simulink model "vdynblksskidpad"  (R2023a)
settings: Solver=ode23tb  StartTime=0.0  StopTime=35  MaxStep=.02  RelTol=1e-1  AbsTol=5e-3
model workspace (MAT data in the model file):
  Eng : object (value not decoded)
  SteerLim = 60
  TrackPoints = [-15 -12 -9 -6 -3 5.58745102111e-16 2.81978007367 5.36354042717 7.38228007367 8.67839071119 9.125 8.67839071119 ... (270 elements, 90x3)]
  Trans : object (value not decoded)
  Ts = 0.02
  VEH : object (value not decoded)
symbols that are objects in the model workspace (value not decoded): Eng, Trans, VEH
undefined symbols (not defined in the file or in its folder): BdyFrm, InertFrm
libraries: autolibsharedcoupling x11, simulink x8, autolibshareddiff x5, sim3dlib x4, autolibutils x3, vehdynlibtirecommon x3, sharedtransform x3, vehdynlibdriver x2, sim3dautolib x2, vehdynlibviscommon x2, visionanalysis x1, vehdynlibtire x1
(part 3 of 3)

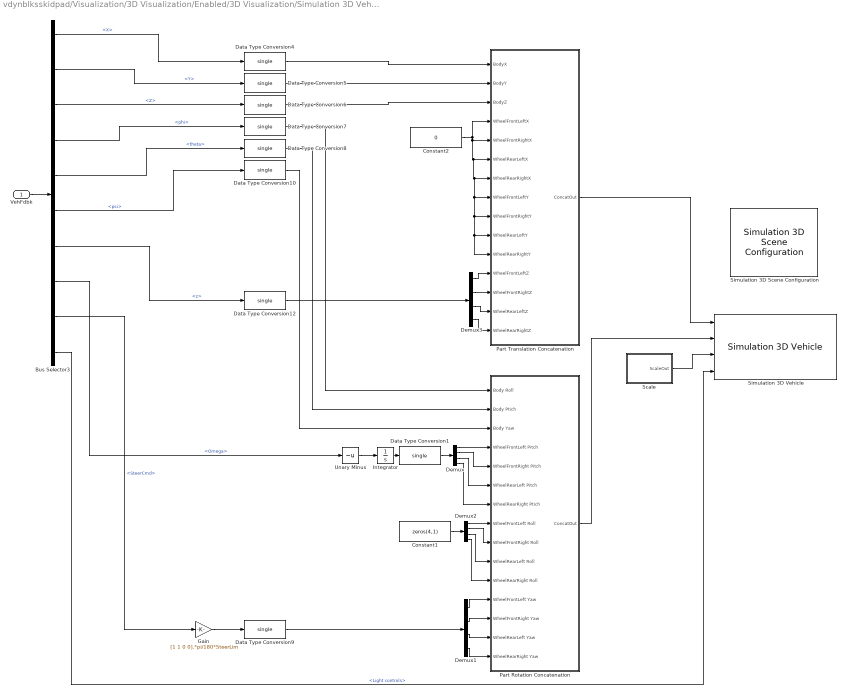
== system vdynblksskidpad/Visualization/3D Visualization/Enabled/3D Visualization/Simulation 3D Vehicle ==
  VehFdbk : Inport
  Bus Selector3 : BusSelector  OutputSignals=VehFdbk.InertFrm.Cg.Disp.X,VehFdbk.InertFrm.Cg.Disp.Y,VehFdbk.InertFrm.Cg.Disp.Z,VehFdbk.InertFrm.Cg.Ang.phi,VehFdbk.InertFrm.Cg.Ang.theta,VehFdbk.InertFrm.Cg.Ang.psi,VehFdbk.Wheels.z,VehFdbk.Wheels.Omega,Driver.SteerCmd,Driver.Light controls
  Constant1 : Constant  Value=zeros(4,1)  OutDataTypeStr=single
  Constant2 : Constant  Value=0  OutDataTypeStr=single
  Data Type Conversion{1,4..10,12} (9 alike) : DataTypeConversion  OutDataTypeStr=single  SaturateOnIntegerOverflow=off  RndMeth=Floor
  Demux{,1..3} (4 alike) : Demux
  Gain : Gain  Gain=[1 1 0 0].*pi/180*SteerLim
  Integrator : Integrator  WrapState=on  WrappedStateUpperValue=2*pi  WrappedStateLowerValue=0  ZeroCross=off
  Part Rotation Concatenation : Subsystem
  Part Translation Concatenation : Subsystem
  Scale : Subsystem
  Simulation 3D Scene Configuration : sim3dlib/Simulation 3D Scene Configuration  Priority=0  ProjectFormat=Default Scenes  SceneDesc=Open surface  ProjectName=C:\Program Files\MATLAB\R2023b\toolbox\shared\sim3d_projects\automotive_project_windows\UE\WindowsNoEditor\VehicleSimulation.exe  ScenePath=/Game/Maps/BlackLake  EnableOpenDRIVE=off  vehTagList={'Scene Origin';'Sim3dActor1';'SimulinkVehicle3'}  vehTag=SimulinkVehicle3  FreeCameraInitialTranslation=[0, 0, 0]  FreeCameraDefaultInitialTranslation=[-6, 0, 2]  FreeCameraInitialRotation=[0, 0, 0]  FreeCameraDefaultInitialRotation=[0, -15, 0]  OpVisEn=off  Ts=Ts  EnableWindow=on  EnableRemoteAccess=off  EnableWeather=off  SunAltitude=40.0  SunAzimuth=90  clouds=10  wind=1  fog=0  rain=0  EnableGeospatial=off  OriginHeight=200  OriginLatitude=40.744652  OriginLongitude=-73.988864  MapStyle=Aerial  AdditionalAssetIDs=[]  UseAdvancedSunSky=off  SolarTime=11  TimeZone=-5  Day=21  Month=9  Year=2022  UseDaylightSavingTime=on  DSTStartDay=10  DSTStartMonth=3  DSTEndDay=3  DSTEndMonth=11  DSTSwitchHour=2  sensorTag=MainCamera3  sensorId=3  sensorName=MainCamera3  mountLoc=Origin  offsetFlag=off  tmountOffset=[0, 0, 0]  rmountOffset=[0, 0, 0]  HorizontalResolution=1280  VerticalResolution=720  HorizontalFOV=60  mountPoint=[0 0 0]  mountOrientation=[0 0 0]  aMode=2  ID=3  GeoTrigger=Inactive
      settings: LibrarySourceBlock=vdynlib/Vehicle Scenarios/Sim3D/Sim3D Core/Simulation 3D Scene Configuration
  Simulation 3D Vehicle : sim3dautolib/Simulation 3D Vehicle  Priority=-1  PassVehMesh=Formula student vehicle  MeshPath=/MathWorksSimulation/Vehicles/Muscle/Meshes/SK_MuscleCar.SK_MuscleCar  VehColor=Red  ActorName=SimulinkVehicle3  VehLightsControl=on  HeadlightColor=[ 1, 1, 1 ]  HighBeamIntensity=100000  LowBeamIntensity=60000  HighBeamConeAngle=1.22  LowBeamConeAngle=1.22  LeftHeadlightOrientation=[ 0, 0 ]  RightHeadlightOrientation=[ 0, 0 ]  BrakelightIntensity=500  ReverselightIntensity=500  SignallightIntensity=500  SignallightPeriod=1  SignalPulseWidth=50  Translation=[ VEH.InitialLongPosition, VEH.InitialLatPosition, VEH.InitialVertPosition *0; zeros(4,3)]  Rotation=[VEH.InitialRollAngle VEH.InitialPitchAngle VEH.InitialYawAngle; zeros( 4, 3 )]  Scale=ones( 5, 3 )  SampleTime=Ts  ActorType=SimulinkVehicle  ID=3  aMode=2  ActorTag=SimulinkVehicle3
      settings: LibrarySourceBlock=vdynlib/Vehicle Scenarios/Sim3D/Sim3D Vehicle/Components/Simulation 3D Vehicle
  Unary Minus : UnaryMinus
  wires:
  Bus Selector3/6 -> Data Type Conversion10/1  "<psi>"
  Bus Selector3/10 -> Simulation 3D Vehicle/4  "<Light controls>"
  Bus Selector3/2 -> Data Type Conversion5/1  "<Y>"
  VehFdbk/1 -> Bus Selector3/1
  Bus Selector3/1 -> Data Type Conversion4/1  "<X>"
  Data Type Conversion10/1 -> Part Rotation Concatenation/3(Body Yaw)
  Data Type Conversion5/1 -> Part Translation Concatenation/2(BodyY)
  Constant2/1 -> Part Translation Concatenation/5(WheelFrontRightX), Part Translation Concatenation/6(WheelRearLeftX), Part Translation Concatenation/7(WheelRearRightX), Part Translation Concatenation/8(WheelFrontLeftY), Part Translation Concatenation/9(WheelFrontRightY), Part Translation Concatenation/10(WheelRearLeftY), Part Translation Concatenation/11(WheelRearRightY), Part Translation Concatenation/4(WheelFrontLeftX)
  Data Type Conversion8/1 -> Part Rotation Concatenation/2(Body Ptich)
  Demux2/2 -> Part Rotation Concatenation/9(WheelFrontRight Roll)
  Demux1/3 -> Part Rotation Concatenation/14(WheelRearLeft Yaw)
  Demux/3 -> Part Rotation Concatenation/6(WheelRearLeft Pitch)
  Data Type Conversion9/1 -> Demux1/1
  Demux1/2 -> Part Rotation Concatenation/13(WheelFrontRight Yaw)
  Demux/2 -> Part Rotation Concatenation/5(WheelFrontRight Pitch)
  Demux2/3 -> Part Rotation Concatenation/10(WheelRearLeft Roll)
  Bus Selector3/5 -> Data Type Conversion8/1  "<theta>"
  Data Type Conversion7/1 -> Part Rotation Concatenation/1(Body Roll)
  Demux3/2 -> Part Translation Concatenation/13(WheelFrontRightZ)
  Data Type Conversion4/1 -> Part Translation Concatenation/1(BodyX)
  Integrator/1 -> Data Type Conversion1/1
  Demux2/1 -> Part Rotation Concatenation/8(WheelFrontLeft Roll)
  Demux1/4 -> Part Rotation Concatenation/15(WheelRearRight Yaw)
  Demux3/4 -> Part Translation Concatenation/15(WheelRearRightZ)
  Bus Selector3/4 -> Data Type Conversion7/1  "<phi>"
  Bus Selector3/7 -> Data Type Conversion12/1  "<z>"
  Bus Selector3/8 -> Unary Minus/1  "<Omega>"
  Data Type Conversion1/1 -> Demux/1
  Constant1/1 -> Demux2/1
  Demux3/3 -> Part Translation Concatenation/14(WheelRearLeftZ)
  Part Rotation Concatenation/1(ConcatOut) -> Simulation 3D Vehicle/2
  Demux3/1 -> Part Translation Concatenation/12(WheelFrontLeftZ)
  Part Translation Concatenation/1(ConcatOut) -> Simulation 3D Vehicle/1
  Demux/1 -> Part Rotation Concatenation/4(WheelFrontLeft Pitch)
  Demux1/1 -> Part Rotation Concatenation/12(WheelFrontLeft Yaw)
  Data Type Conversion6/1 -> Part Translation Concatenation/3(BodyZ)
  Unary Minus/1 -> Integrator/1
  Demux/4 -> Part Rotation Concatenation/7(WheelRearRight Ptich)
  Demux2/4 -> Part Rotation Concatenation/11(WheelRearRight Roll)
  Data Type Conversion12/1 -> Demux3/1
  Scale/1(ScaleOut) -> Simulation 3D Vehicle/3
  Bus Selector3/3 -> Data Type Conversion6/1  "<Z>"
  Bus Selector3/9 -> Gain/1  "<SteerCmd>"
  Gain/1 -> Data Type Conversion9/1

== system vdynblksskidpad/Visualization/3D Visualization/Enabled/Cones/Disabled ==

== system vdynblksskidpad/Visualization/3D Visualization/Enabled/Cones/Enabled ==
  Simulation 3D Actor : sim3dlib/Simulation 3D Actor  ActorName=Sim3dActor1  ParentName=Scene Origin  Operation=Create at setup  InitScriptText=|  SampleTime=Ts  Translation=single([0 0 0])  Rotation=single([0 0 0])  Scale=single([1 1 1])  aMode=5  ActorTag=Sim3dActor1  ActorType=Sim3dActor  ID=1
      | entryWidth =3.453;
      | conesZ0 = 0;
      | entryConesLoc = [entryWidth/2 -12;...
      |                  -entryWidth/2 -12;...
      |                  -entryWidth/2 -10;...
      |                  entryWidth/2 -10];
      | entryConesLoc= fliplr(entryConesLoc); % account for game engine coords
      | rightInnerRingLoc = [entryWidth/2 0;...%1
      |                   4.58/2 -2.834;...%2
      |                   7.787/2 -5.231;...%3
      |                   12.588/2 -6.835;...%4
      |                   18.25/2 -7.398;...%5
      |                   23.912/2 -6.835;...%6
      |                   28.713/2 -5.231;...%7
      |                   31.92/2 -2.834;...%8
      |                   33.047/2 0;...%9
      |                   31.92/2 2.834;...%10
      |                   28.713/2 5.231;...%11
      |                   23.912/2 6.835;...%12
      |                   18.25/2 7.398;...%13
      |                   12.588/2 6.835;...%14
      |                   7.787/2 5.231;...%15
      |                   4.58/2 2.834;...%16    
      |                   ];
      | rightInnerRingLoc = fliplr(rightInnerRingLoc);
      | leftInnerRingLoc = rightInnerRingLoc.*[1 -1];
      | rightOutterRingLoc = [entryWidth/2 7.939;...% right side entry to exit zone
      |                       9.945/2 10.026;...
      |                       18.25/2 10.852;...
      |                       26.555/2 10.026;...
      |                       33.596/2 7.673;...
      |                       38.301/2 4.153;...
      |                       39.953/2 0;...
      |                       38.301/2 -4.153;...
      |                       33.596/2 -7.673;...
      |                       26.555/2 -10.026;...
      |                       18.25/2 -10.852;...
      |                       9.945/2 -10.026;...                      
      |                       entryWidth/2 -7.939;...% right side after entry zone                      
      |                       ];
      | rightOutterRingLoc = fliplr(rightOutterRingLoc);
      | leftOutterRingLoc = rightOutterRingLoc.*[1 -1];
      | 
      | exitConesLoc = [entryWidth/2 16;...
      |                  -entryWidth/2 16;...
      |                  entryWidth/2-1 16;...
      |                  -entryWidth/2+1 16;...
      |                  -entryWidth/2 14;...
      |                  entryWidth/2 14;...
      |                  -entryWidth/2 12;...
      |                  entryWidth/2 12;...
      |                  -entryWidth/2 10;...
      |                  entryWidth/2 10];
      | exitConesLoc= fliplr(exitConesLoc); % account for game engine coords
      | 
      | timeConesLoc = fliplr([entryWidth/2 .5;...
      |                  -entryWidth/2 .5;...
      |                  entryWidth/2 -.5;...
      |                  -entryWidth/2 -.5]);
      | 
      | blueCones = [rightOutterRingLoc; leftInnerRingLoc];
      | yellowCones = [rightInnerRingLoc; leftOutterRingLoc];
      | smallOrangeCones = [entryConesLoc; exitConesLoc];
      | largeOrangeCones = timeConesLoc;
      | 
      | skidSurface = sim3d.Actor('ActorName','BaseSurface');
      | skidSurface.createShape('box',[45,45,+0.03]);
      | skidSurface.Color = [68 68 71]./100;
      | skidSurface.Translation = [0 0 0]; 
      | skidSurface.Texture = fullfile(pwd,"vdynskidpad.png"); 
      | skidSurface.TextureTransform.Scale = [1 1];
      | skidSurface.TextureTransform.Angle = 0;
      | skidSurface.Shininess = 0;
      | skidSurface.Transparency = 0;
      | skidSurface.TextureMapping.Blend = 1;
      | skidSurface.TextureMapping.Roughness = .8;
      | World.add(skidSurface,Actor);
      | 
      | nCones = length(largeOrangeCones);
      | for coneNum = 1:nCones    
      |     coneName = "LCone_" + num2str(coneNum);
      |     conLoc = [largeOrangeCones(coneNum,:) conesZ0];
      |     cone = sim3d.Actor('ActorName',coneName,'Mesh','/Game/Environment/Industrial/Props/Cone/Mesh/SM_Cone.SM_Cone',...
      |         'Mobility', sim3d.utils.MobilityTypes.Movable,...
      |         'SimulatePhysics', true,...
      |         'Translation',conLoc,...
      |         'EnableGravity', true);    
      |     %cone.Shadows = true;
      |     World.add(cone,Actor);
      | end
      | 
      | smallCones = [blueCones; yellowCones; smallOrangeCones]; 
      | for coneNum = 1:length(smallCones)    
      |     coneName = "sCone_" + num2str(coneNum);
      |     conLoc = [smallCones(coneNum,:) conesZ0];
      |     cone = sim3d.Actor('ActorName',coneName,'Mesh','/Game/Environment/Industrial/Props/Cone/Mesh/SM_Cone.SM_Cone',...
      |         'Mobility', sim3d.utils.MobilityTypes.Movable,...
      |         'SimulatePhysics', true,...
      |         'Translation',conLoc,...
      |         'EnableGravity', true,...
      |         'Scale',ones(1,3).*325/500);    
      |     cone.Color= [102 140 204]./255;
      |     World.add(cone,Actor);
      | end
      settings: LibrarySourceBlock=sl3dlib/Simulation 3D/Simulation 3D Actor
  Terminator : Terminator
  wires:
  Simulation 3D Actor/1 -> Terminator/1

== system vdynblksskidpad/Formula Student Vehicle/Simulink Physics - 7DOF/Powertrain & Driveline/Brakes and Wheels/Tire2Veh/Wheel Angles ==
  Front : Inport
  Camber : Inport  Port=2
  Constant : Constant  Value=zeros(4,1)
  Reshape : Reshape  OutputDimensionality=Row vector (2-D)
  Reshape1 : Reshape  OutputDimensionality=Row vector (2-D)
  Reshape2 : Reshape  OutputDimensionality=Row vector (2-D)
  Vector Concatenate3 : Concatenate  NumInputs=3  Mode=Multidimensional array
  Vehicle : Outport  VectorParamsAs1DForOutWhenUnconnected=off
  wires:
  Reshape/1 -> Vector Concatenate3/3
  Reshape2/1 -> Vector Concatenate3/2
  Vector Concatenate3/1 -> Vehicle/1
  Reshape1/1 -> Vector Concatenate3/1
  Front/1 -> Reshape/1
  Camber/1 -> Reshape1/1
  Constant/1 -> Reshape2/1

== system vdynblksskidpad/Formula Student Vehicle/Simulink Physics - 7DOF/Powertrain & Driveline/Brakes and Wheels/Tire2Veh/Wheel to Body Transform ==
  Forces : Inport  PortDimensions=[3,1]  Partition=on  PartitionDimension=2  PartitionWidth=1  PartitionOffset=0
  WheelAngles : Inport  Port=2  Partition=on  PartitionDimension=2  PartitionWidth=1  PartitionOffset=0
  Constant : Constant  Value=[pi;0;0]
  Demux1 : Demux  Outputs=3
  Divide1 : Product  Inputs=***  Multiplication=Matrix(*)
  For Each : ForEach  DisableCoverage=on
  Rotation Angles to Direction Cosine Matrix : sharedtransform/Rotation Angles to Direction Cosine Matrix  rotationOrder=ZYX  aMode=2
  Rotation Angles to Direction Cosine Matrix1 : sharedtransform/Rotation Angles to Direction Cosine Matrix  rotationOrder=ZYX  aMode=2
  Selector : Selector  InputPortWidth=3  IndexOptions=Index vector (dialog)  Indices=[3 2 1]  OutputSizes=1
  Selector1 : Selector  InputPortWidth=3  IndexOptions=Index vector (dialog)  Indices=[3 2 1]  OutputSizes=1
  Transpose : Math  Operator=transpose
  Fx : Outport  ConcatenationDimension=1  VectorParamsAs1DForOutWhenUnconnected=off
  Fy : Outport  Port=2  ConcatenationDimension=1  VectorParamsAs1DForOutWhenUnconnected=off
  Fz : Outport  Port=3  ConcatenationDimension=1  VectorParamsAs1DForOutWhenUnconnected=off
  wires:
  Demux1/1 -> Fx/1
  Demux1/2 -> Fy/1
  Demux1/3 -> Fz/1
  Rotation Angles to Direction Cosine Matrix/1 -> Transpose/1
  Forces/1 -> Divide1/3
  WheelAngles/1 -> Selector/1
  Selector/1 -> Rotation Angles to Direction Cosine Matrix/1
  Rotation Angles to Direction Cosine Matrix1/1 -> Divide1/2
  Divide1/1 -> Demux1/1
  Selector1/1 -> Rotation Angles to Direction Cosine Matrix1/1
  Constant/1 -> Selector1/1
  Transpose/1 -> Divide1/1

== system vdynblksskidpad/Formula Student Vehicle/Simulink Physics - 7DOF/Powertrain & Driveline/Brakes and Wheels/Veh2Tire/Wheel to Body Transform ==
  VelVeh : Inport  Partition=on  PartitionDimension=2  PartitionWidth=1  PartitionOffset=0
  WhlAng : Inport  Port=2  Partition=on  PartitionDimension=2  PartitionWidth=1  PartitionOffset=0
  Demux1 : Demux  Outputs=3
  Divide1 : Product  Inputs=**  Multiplication=Matrix(*)
  For Each : ForEach  DisableCoverage=on
  Rotation Angles to Direction Cosine Matrix : sharedtransform/Rotation Angles to Direction Cosine Matrix  rotationOrder=ZYX  aMode=2
  Selector : Selector  InputPortWidth=3  IndexOptions=Index vector (dialog)  Indices=[3 2 1]  OutputSizes=1
  xdotWheel : Outport  ConcatenationDimension=1  VectorParamsAs1DForOutWhenUnconnected=off
  ydotWheel : Outport  Port=2  ConcatenationDimension=1  VectorParamsAs1DForOutWhenUnconnected=off
  zdotWheel : Outport  Port=3  ConcatenationDimension=1  VectorParamsAs1DForOutWhenUnconnected=off
  wires:
  Divide1/1 -> Demux1/1
  Demux1/1 -> xdotWheel/1
  Demux1/2 -> ydotWheel/1
  Demux1/3 -> zdotWheel/1
  Rotation Angles to Direction Cosine Matrix/1 -> Divide1/1
  VelVeh/1 -> Divide1/2
  WhlAng/1 -> Selector/1
  Selector/1 -> Rotation Angles to Direction Cosine Matrix/1

== system vdynblksskidpad/Formula Student Vehicle/Simulink Physics - 7DOF/Powertrain & Driveline/Powertrain/Transmission/Ideal ==
  GearCmd : Inport
  EngTrq : Inport  Port=2
  PropShftSpd : Inport  Port=3
  Ideal Fixed Gear Transmission : autolibsharedtransfixedgear/Ideal Fixed Gear Transmission  VariantControl=0  TransEffModelPopup=Gear only  gearInterp=Linear point-slope  G=Trans.GearNums  Trq_bpts=[25, 50, 75, 100, 150, 200, 250]  omega_bpts=[52.4 78.5 105 131 157 183 209 262 314 419 524]  Temp_bpts=[313 358]  N=Trans.GearRatios  Jout=Trans.Inertias  bout=Trans.DampingCoeffs  eta=Trans.Efficiencies  eta_tbl=reshape([0.53 0.71 0.77 0.79 0.82 0.82 0.82 0.5 0.7 0.77 0.79 0.82 0.82 0.82 0.54 0.72 0.78 0.81 0.83 0.82 0.82 0.56 0.73 0.79 0.81 0.84 0.82 0.82 0.58 0.74 0.79 0.82 0.84 0.82 0.82 0.57 0.74 0.79 0.82 0.84 0.82 0.82 0.58 0.74 0.79 0.82 0.84 0.82 0.82 0.58 0.74 0.79 0.82 0.84 0.82 0.82 0.57 0.74 0.8 0.82 0.85 0.82 0.82 0.55 0.73 0.78 0.81 0.84 0.82 0.82 0.51 0.71 0.77 0.81 0.84 0.82 0.82 0.53 0.71 0.77 0.79 0.82 0.82 0.82 0.5 0.7 0.77 0.79 0.82 0.82 0.82 0.54 0.72 0.78 0.81 0.83 0.82 0.82 0.56 0.73 0.79 0.81 0.84 0.82 0.82 0.58 0.74 0.79 0.82 0.84 0.82 0.82 0.57 0.74 0.79 0.82 0.84 0.82 0.82 0.58 0.74 0.79 0.82 0.84 0.82 0.82 0.58 0.74 0.79 0.82 0.84 0.82 0.82 0.57 0.74 0.8 0.82 0.85 0.82 0.82 0.55 0.73 0.78 0.81 0.84 0.82 0.82 0.51 0.71 0.77 0.81 0.84 0.82 0.82 0.53 0.71 0.77 0.79 0.82 0.82 0.82 0.5 0.7 0.77 0.79 0.82 0.82 0.82 0.54 0.72 0.78 0.81 0.83 0.82 0.82 0.56 0.73 0.79 0.81 0.84 0.82 0.82 0.58 0.74 0.79 0.82 0.84 0.82 0.82 0.57 0.74 0.79 0.82 0.84 0.82 0.82 0.58 0.74 0.79 0.82 0.84 0.82 0.82 0.58 0.74 0.79 0.82 0.84 0.82 0.82 0.57 0.74 0.8 0.82 0.85 0.82 0.82 0.55 0.73 0.78 0.81 0.84 0.82 0.82 0.51 0.71 0.77 0.81 0.84 0.82 0.82 0.7 0.79 0.82 0.83 0.84 0.84 0.84 0.63 0.76 0.8 0.82 0.83 0.84 0.84 0.58 0.74 0.79 0.81 0.83 0.84 0.84 0.58 0.74 0.79 0.81 0.83 0.84 0.84 0.58 0.74 0.79 0.81 0.84 0.84 0.84 0.57 0.73 0.78 0.81 0.84 0.85 0.84 0.57 0.73 0.79 0.81 0.84 0.85 0.84 0.56 0.73 0.78 0.81 0.83 0.85 0.84 0.55 0.73 0.78 0.81 0.84 0.85 0.84 0.52 0.71 0.77 0.8 0.83 0.85 0.84 0.48 0.69 0.76 0.79 0.83 0.84 0.84 0.64 0.76 0.8 0.81 0.83 0.84 0.84 0.56 0.73 0.78 0.8 0.83 0.84 0.84 0.54 0.71 0.77 0.8 0.82 0.84 0.84 0.53 0.71 0.77 0.8 0.83 0.84 0.84 0.51 0.71 0.77 0.8 0.83 0.84 0.85 0.52 0.7 0.77 0.8 0.83 0.84 0.85 0.51 0.71 0.76 0.79 0.83 0.84 0.85 0.5 0.69 0.76 0.79 0.82 0.84 0.85 0.45 0.68 0.75 0.78 0.82 0.84 0.85 0.43 0.67 0.74 0.78 0.81 0.83 0.84 0.38 0.63 0.71 0.75 0.8 0.82 0.83 0.65 0.79 0.84 0.85 0.88 0.89 0.89 0.56 0.75 0.81 0.83 0.86 0.88 0.89 0.52 0.72 0.79 0.83 0.86 0.88 0.88 0.51 0.72 0.79 0.83 0.86 0.88 0.89 0.49 0.71 0.78 0.82 0.86 0.88 0.89 0.47 0.7 0.78 0.82 0.86 0.87 0.88 0.45 0.69 0.77 0.81 0.85 0.87 0.88 0.4 0.67 0.75 0.8 0.84 0.86 0.88 0.3 0.64 0.73 0.78 0.83 0.86 0.87 0.17 0.55 0.67 0.73 0.8 0.83 0.85 0.089 0.45 0.61 0.69 0.77 0.81 0.83 0.61 0.75 0.82 0.84 0.87 0.87 0.88 0.54 0.73 0.8 0.82 0.86 0.87 0.88 0.51 0.71 0.79 0.82 0.86 0.87 0.88 0.52 0.72 0.79 0.82 0.86 0.87 0.89 0.52 0.72 0.8 0.83 0.86 0.88 0.89 0.53 0.72 0.79 0.82 0.86 0.87 0.89 0.5 0.7 0.78 0.82 0.86 0.88 0.88 0.46 0.69 0.77 0.81 0.85 0.87 0.88 0.4 0.67 0.75 0.8 0.83 0.86 0.88 0.33 0.64 0.73 0.78 0.83 0.85 0.87 0.33 0.64 0.73 0.78 0.83 0.85 0.87 0.78 0.85 0.87 0.88 0.89 0.89 0.89 0.73 0.83 0.86 0.88 0.89 0.89 0.89 0.72 0.83 0.86 0.88 0.89 0.89 0.89 0.72 0.83 0.87 0.89 0.9 0.89 0.89 0.72 0.83 0.87 0.88 0.9 0.89 0.89 0.71 0.83 0.87 0.88 0.9 0.89 0.89 0.71 0.83 0.86 0.88 0.9 0.89 0.89 0.7 0.82 0.86 0.88 0.9 0.89 0.89 0.69 0.82 0.86 0.88 0.9 0.89 0.89 0.67 0.81 0.86 0.88 0.9 0.89 0.89 0.63 0.79 0.85 0.87 0.89 0.89 0.89 0.78 0.85 0.87 0.88 0.89 0.89 0.89 0.73 0.83 0.86 0.88 0.89 0.89 0.89 0.72 0.83 0.86 0.88 0.89 0.89 0.89 0.72 0.83 0.87 0.89 0.9 0.89 0.89 0.72 0.83 0.87 0.88 0.9 0.89 0.89 0.71 0.83 0.87 0.88 0.9 0.89 0.89 0.71 0.83 0.86 0.88 0.9 0.89 0.89 0.7 0.82 0.86 0.88 0.9 0.89 0.89 0.69 0.82 0.86 0.88 0.9 0.89 0.89 0.67 0.81 0.86 0.88 0.9 0.89 0.89 0.63 0.79 0.85 0.87 0.89 0.89 0.89 0.78 0.85 0.87 0.88 0.89 0.89 0.89 0.73 0.83 0.86 0.88 0.89 0.89 0.89 0.72 0.83 0.86 0.88 0.89 0.89 0.89 0.72 0.83 0.87 0.89 0.9 0.89 0.89 0.72 0.83 0.87 0.88 0.9 0.89 0.89 0.71 0.83 0.87 0.88 0.9 0.89 0.89 0.71 0.83 0.86 0.88 0.9 0.89 0.89 0.7 0.82 0.86 0.88 0.9 0.89 0.89 0.69 0.82 0.86 0.88 0.9 0.89 0.89 0.67 0.81 0.86 0.88 0.9 0.89 0.89 0.63 0.79 0.85 0.87 0.89 0.89 0.89 0.82 0.87 0.88 0.89 0.89 0.89 0.89 0.81 0.87 0.89 0.89 0.9 0.9 0.89 0.76 0.85 0.87 0.89 0.9 0.89 0.89 0.72 0.83 0.86 0.88 0.89 0.89 0.89 0.72 0.83 0.86 0.88 0.89 0.9 0.89 0.71 0.82 0.86 0.88 0.89 0.9 ...(+1314 chars))  G_o=0  omega_o=0  omegaN_o=0  tau_s=Trans.ShiftTau  maxAbsSpd=5e3  aMode=2
      settings: LibrarySourceBlock=vdynlib/Powertrain/Transmission/Ideal Fixed Gear Transmission
  Prop Shaft : autolibsharedcoupling/Torsional Compliance  port_config=Simulink  extInfo=off  k=5e3  b=10  theta_o=0  domega_o=0  omega_c=100  blkID=0  aMode=2
      settings: LibrarySourceBlock=vdynlib/Powertrain/Drivetrain/Couplings/Torsional Compliance
  Unit Conversion : UnitConversion
  Info : Outport  VectorParamsAs1DForOutWhenUnconnected=off
  EngSpd : Outport  Port=2  VectorParamsAs1DForOutWhenUnconnected=off
  DrvShfTrq : Outport  Port=3  VectorParamsAs1DForOutWhenUnconnected=off
  wires:
  Ideal Fixed Gear Transmission/2 -> Unit Conversion/1
  GearCmd/1 -> Ideal Fixed Gear Transmission/1
  Ideal Fixed Gear Transmission/1 -> Info/1
  PropShftSpd/1 -> Prop Shaft/2
  Ideal Fixed Gear Transmission/3 -> Prop Shaft/1
  Prop Shaft/2 -> DrvShfTrq/1
  Prop Shaft/1 -> Ideal Fixed Gear Transmission/3
  EngTrq/1 -> Ideal Fixed Gear Transmission/2
  Unit Conversion/1 -> EngSpd/1

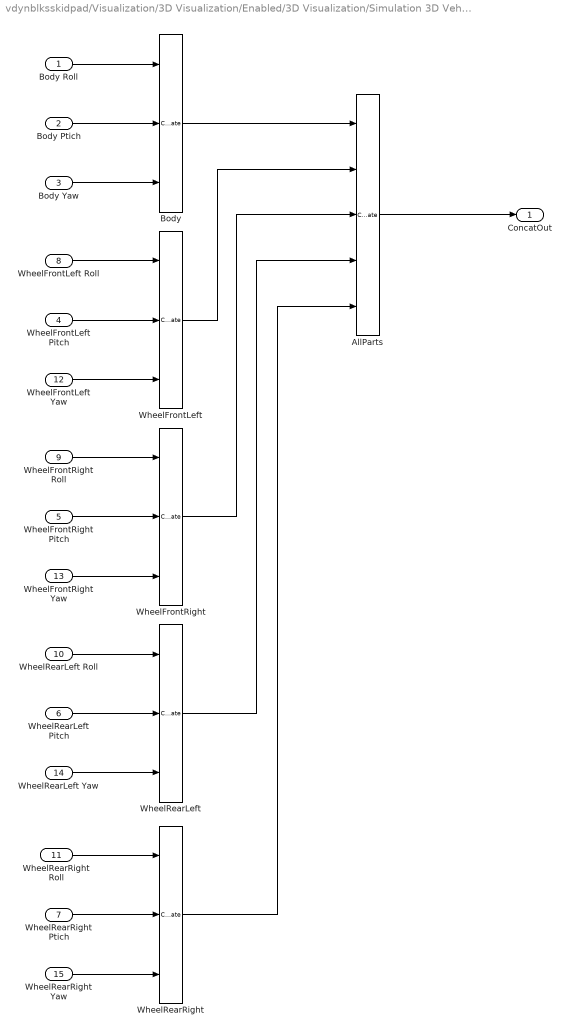
== system vdynblksskidpad/Visualization/3D Visualization/Enabled/3D Visualization/Simulation 3D Vehicle/Part Rotation Concatenation ==
  Body Roll : Inport
  Body Ptich : Inport  Port=2
  Body Yaw : Inport  Port=3
  WheelFrontLeft Pitch : Inport  Port=4
  WheelFrontRight Pitch : Inport  Port=5
  WheelRearLeft Pitch : Inport  Port=6
  WheelRearRight Ptich : Inport  Port=7
  WheelFrontLeft Roll : Inport  Port=8
  WheelFrontRight Roll : Inport  Port=9
  WheelRearLeft Roll : Inport  Port=10
  WheelRearRight Roll : Inport  Port=11
  WheelFrontLeft Yaw : Inport  Port=12
  WheelFrontRight Yaw : Inport  Port=13
  WheelRearLeft Yaw : Inport  Port=14
  WheelRearRight Yaw : Inport  Port=15
  AllParts : Concatenate  NumInputs=5  Mode=Multidimensional array
  Body : Concatenate  NumInputs=3  Mode=Multidimensional array  ConcatenateDimension=2
  WheelFrontLeft : Concatenate  NumInputs=3  Mode=Multidimensional array  ConcatenateDimension=2
  WheelFrontRight : Concatenate  NumInputs=3  Mode=Multidimensional array  ConcatenateDimension=2
  WheelRearLeft : Concatenate  NumInputs=3  Mode=Multidimensional array  ConcatenateDimension=2
  WheelRearRight : Concatenate  NumInputs=3  Mode=Multidimensional array  ConcatenateDimension=2
  ConcatOut : Outport  VectorParamsAs1DForOutWhenUnconnected=off
  wires:
  Body Yaw/1 -> Body/3
  WheelFrontLeft Yaw/1 -> WheelFrontLeft/3
  WheelFrontLeft/1 -> AllParts/2
  Body/1 -> AllParts/1
  WheelRearLeft/1 -> AllParts/4
  WheelFrontRight/1 -> AllParts/3
  WheelRearRight Yaw/1 -> WheelRearRight/3
  WheelRearLeft Yaw/1 -> WheelRearLeft/3
  AllParts/1 -> ConcatOut/1
  WheelRearRight/1 -> AllParts/5
  WheelFrontRight Yaw/1 -> WheelFrontRight/3
  Body Ptich/1 -> Body/2
  Body Roll/1 -> Body/1
  WheelFrontLeft Pitch/1 -> WheelFrontLeft/2
  WheelFrontLeft Roll/1 -> WheelFrontLeft/1
  WheelFrontRight Pitch/1 -> WheelFrontRight/2
  WheelFrontRight Roll/1 -> WheelFrontRight/1
  WheelRearLeft Pitch/1 -> WheelRearLeft/2
  WheelRearLeft Roll/1 -> WheelRearLeft/1
  WheelRearRight Ptich/1 -> WheelRearRight/2
  WheelRearRight Roll/1 -> WheelRearRight/1

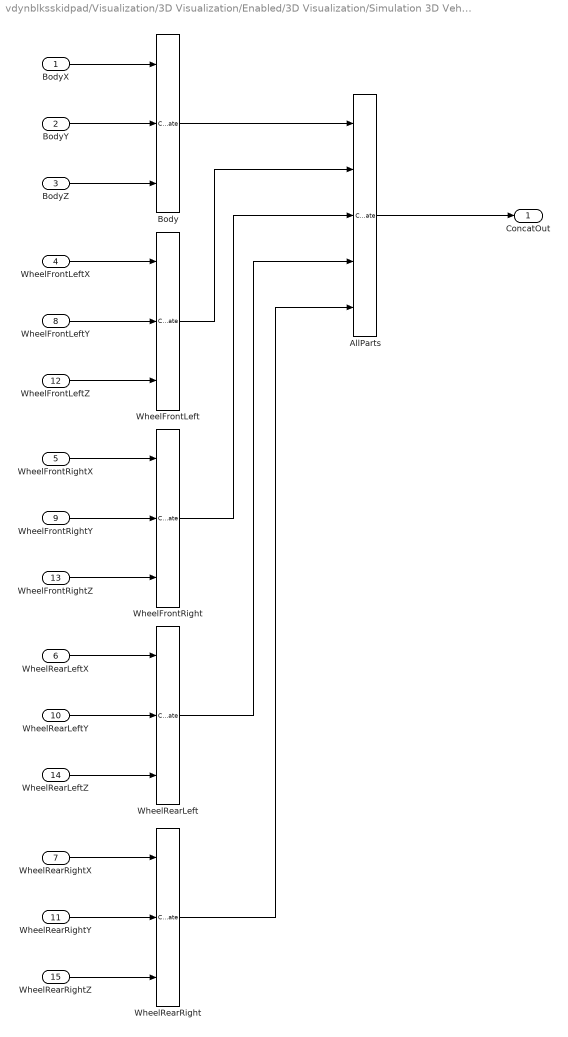
== system vdynblksskidpad/Visualization/3D Visualization/Enabled/3D Visualization/Simulation 3D Vehicle/Part Translation Concatenation ==
  BodyX : Inport
  BodyY : Inport  Port=2
  BodyZ : Inport  Port=3
  WheelFrontLeftX : Inport  Port=4
  WheelFrontRightX : Inport  Port=5
  WheelRearLeftX : Inport  Port=6
  WheelRearRightX : Inport  Port=7
  WheelFrontLeftY : Inport  Port=8
  WheelFrontRightY : Inport  Port=9
  WheelRearLeftY : Inport  Port=10
  WheelRearRightY : Inport  Port=11
  WheelFrontLeftZ : Inport  Port=12
  WheelFrontRightZ : Inport  Port=13
  WheelRearLeftZ : Inport  Port=14
  WheelRearRightZ : Inport  Port=15
  AllParts : Concatenate  NumInputs=5  Mode=Multidimensional array
  Body : Concatenate  NumInputs=3  Mode=Multidimensional array  ConcatenateDimension=2
  WheelFrontLeft : Concatenate  NumInputs=3  Mode=Multidimensional array  ConcatenateDimension=2
  WheelFrontRight : Concatenate  NumInputs=3  Mode=Multidimensional array  ConcatenateDimension=2
  WheelRearLeft : Concatenate  NumInputs=3  Mode=Multidimensional array  ConcatenateDimension=2
  WheelRearRight : Concatenate  NumInputs=3  Mode=Multidimensional array  ConcatenateDimension=2
  ConcatOut : Outport  VectorParamsAs1DForOutWhenUnconnected=off
  wires:
  BodyX/1 -> Body/1
  BodyZ/1 -> Body/3
  WheelFrontLeftX/1 -> WheelFrontLeft/1
  WheelFrontLeftZ/1 -> WheelFrontLeft/3
  WheelFrontLeftY/1 -> WheelFrontLeft/2
  BodyY/1 -> Body/2
  WheelFrontLeft/1 -> AllParts/2
  WheelRearRightX/1 -> WheelRearRight/1
  Body/1 -> AllParts/1
  WheelRearLeft/1 -> AllParts/4
  WheelFrontRight/1 -> AllParts/3
  WheelRearRightZ/1 -> WheelRearRight/3
  WheelFrontRightY/1 -> WheelFrontRight/2
  WheelFrontRightX/1 -> WheelFrontRight/1
  WheelRearRightY/1 -> WheelRearRight/2
  WheelRearLeftZ/1 -> WheelRearLeft/3
  AllParts/1 -> ConcatOut/1
  WheelRearLeftY/1 -> WheelRearLeft/2
  WheelRearRight/1 -> AllParts/5
  WheelRearLeftX/1 -> WheelRearLeft/1
  WheelFrontRightZ/1 -> WheelFrontRight/3

== system vdynblksskidpad/Visualization/3D Visualization/Enabled/3D Visualization/Simulation 3D Vehicle/Scale ==
  Constant{1..12,17,32..33} (15 alike) : Constant  OutDataTypeStr=single
  PartConcatenation : Subsystem
  ScaleOut : Outport  VectorParamsAs1DForOutWhenUnconnected=off
  wires:
  Constant10/1 -> PartConcatenation/15(WheelRearRightZ)
  Constant9/1 -> PartConcatenation/14(WheelRearRightY)
  Constant11/1 -> PartConcatenation/13(WheelRearRightX)
  Constant7/1 -> PartConcatenation/12(WheelRearLeftZ)
  Constant6/1 -> PartConcatenation/11(WheelRearLeftY)
  Constant8/1 -> PartConcatenation/10(WheelRearLeftX)
  Constant4/1 -> PartConcatenation/9(WheelFrontRightZ)
  Constant3/1 -> PartConcatenation/8(WheelFrontRightY)
  Constant5/1 -> PartConcatenation/7(WheelFrontRightX)
  Constant2/1 -> PartConcatenation/6(WheelFrontLeftZ)
  Constant1/1 -> PartConcatenation/5(WheelFrontLeftY)
  Constant33/1 -> PartConcatenation/4(WheelFrontLeftX)
  Constant32/1 -> PartConcatenation/3(BodyZ)
  Constant17/1 -> PartConcatenation/2(BodyY)
  Constant12/1 -> PartConcatenation/1(BodyX)
  PartConcatenation/1(ConcatOut) -> ScaleOut/1

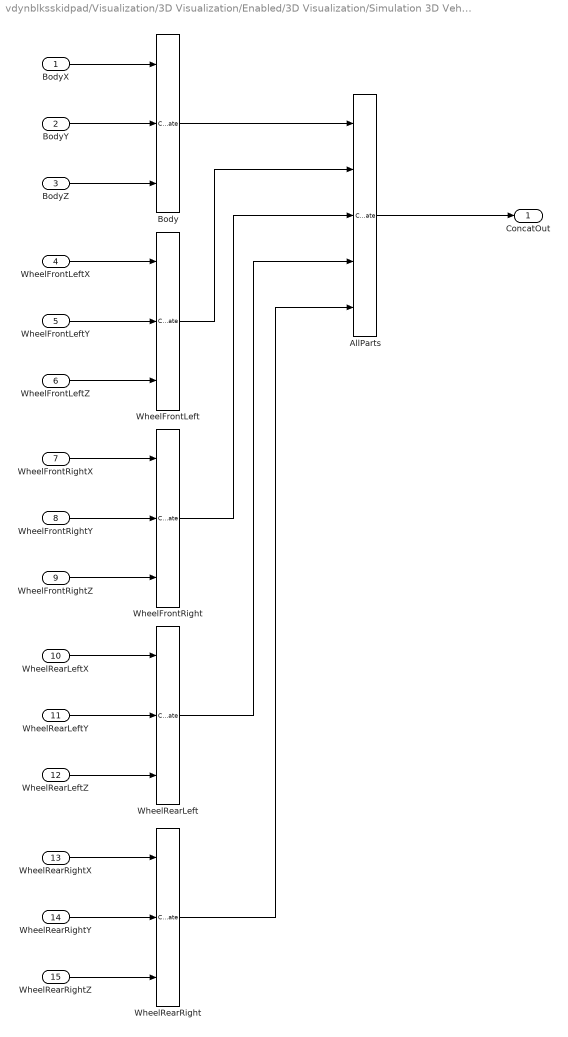
== system vdynblksskidpad/Visualization/3D Visualization/Enabled/3D Visualization/Simulation 3D Vehicle/Scale/PartConcatenation ==
  BodyX : Inport
  BodyY : Inport  Port=2
  BodyZ : Inport  Port=3
  WheelFrontLeftX : Inport  Port=4
  WheelFrontLeftY : Inport  Port=5
  WheelFrontLeftZ : Inport  Port=6
  WheelFrontRightX : Inport  Port=7
  WheelFrontRightY : Inport  Port=8
  WheelFrontRightZ : Inport  Port=9
  WheelRearLeftX : Inport  Port=10
  WheelRearLeftY : Inport  Port=11
  WheelRearLeftZ : Inport  Port=12
  WheelRearRightX : Inport  Port=13
  WheelRearRightY : Inport  Port=14
  WheelRearRightZ : Inport  Port=15
  AllParts : Concatenate  NumInputs=5  Mode=Multidimensional array
  Body : Concatenate  NumInputs=3  Mode=Multidimensional array  ConcatenateDimension=2
  WheelFrontLeft : Concatenate  NumInputs=3  Mode=Multidimensional array  ConcatenateDimension=2
  WheelFrontRight : Concatenate  NumInputs=3  Mode=Multidimensional array  ConcatenateDimension=2
  WheelRearLeft : Concatenate  NumInputs=3  Mode=Multidimensional array  ConcatenateDimension=2
  WheelRearRight : Concatenate  NumInputs=3  Mode=Multidimensional array  ConcatenateDimension=2
  ConcatOut : Outport  VectorParamsAs1DForOutWhenUnconnected=off
  wires:
  BodyX/1 -> Body/1
  BodyZ/1 -> Body/3
  WheelFrontLeftX/1 -> WheelFrontLeft/1
  WheelFrontLeftZ/1 -> WheelFrontLeft/3
  WheelFrontLeftY/1 -> WheelFrontLeft/2
  BodyY/1 -> Body/2
  WheelFrontLeft/1 -> AllParts/2
  WheelRearRightX/1 -> WheelRearRight/1
  Body/1 -> AllParts/1
  WheelRearLeft/1 -> AllParts/4
  WheelFrontRight/1 -> AllParts/3
  WheelRearRightZ/1 -> WheelRearRight/3
  WheelFrontRightY/1 -> WheelFrontRight/2
  WheelFrontRightX/1 -> WheelFrontRight/1
  WheelRearRightY/1 -> WheelRearRight/2
  WheelRearLeftZ/1 -> WheelRearLeft/3
  AllParts/1 -> ConcatOut/1
  WheelRearLeftY/1 -> WheelRearLeft/2
  WheelRearRight/1 -> AllParts/5
  WheelRearLeftX/1 -> WheelRearLeft/1
  WheelFrontRightZ/1 -> WheelFrontRight/3

== matlab function vdynblksskidpad/Skidpad Reference/Lap Time Counter ==
  settings: updateMethod=DISCRETE
  data: X input; LapTimes output; Y input; psi input; t input; CurrLapNum output
function [LapTimes, CurrLapNum]  = laptimer(X, Y, psi, t)
% A very simple lap counter. Assumes the start line is at X = 0, along Y
% axis within a specified track width
%
% Copyright 2022 The MathWorks, Inc.
%
%#codegen
coder.allowpcode('plain')
NLaps = 4;
trackWidth = 3.5; 
[LapTimes, CurrLapNum] = vdynlaptimer(X, Y, psi, t,NLaps,trackWidth);
end

== matlab function vdynblksskidpad/MATLAB Function1 ==
  data: bboxes input; labels input; outImg output; img input
function outImg = AnnotateImage(bboxes, labels, img)
    % Annotate detections in the image. 

    if ~isempty(bboxes)
        for i = 1:numel(labels)
            img = insertObjectAnnotation(img, "rectangle", bboxes(i, :), char(labels(i)));
        end
    end

    outImg = img;

end
